simulink model "VC_GFM"  (R2023b)
settings: Solver=FixedStepAuto  StartTime=0.0  StopTime=1.5  RelTol=1e-3
InitFcn:
  | % 1. Récupérer les valeurs directement depuis le masque du Load Flow Bus4
  | V_amplitude_pu = str2double(get_param([bdroot '/Load Flow Bus4'], 'VLF'));
  | V_phase_deg    = str2double(get_param([bdroot '/Load Flow Bus4'], 'angleLF'));
  | 
  | % Assurez-vous que Vn est bien défini dans le modèle ou définissez-le ici
  | % Vn = 400; % (Exemple, à décommenter et adapter si Vn n'est pas connu du modèle)
  | 
  | % 2. Calculer et formater la chaîne de caractères pour le Sequence Analyzer
  | InInit_str = ['[', ...
  |     num2str(V_amplitude_pu * Vn * sqrt(2), '%.6f'), ', ', ...
  |     num2str(V_phase_deg, '%.6f'), ']'];
  | InInit_str2 = ['[', ...
  |     num2str((sqrt(2) * 0.5 * Sn_vcGFM) / (3 * V_amplitude_pu * Vn), '%.6f'), ', ', ...
  |     '0]'];
  | 
  | % 3. Injecter la valeur dans le Sequence Analyzer
  | set_param([bdroot '/Sequence Analyzer'], 'InInit', InInit_str);
  | set_param([bdroot '/Sequence Analyzer1'], 'InInit', InInit_str2);
undefined symbols (not defined in the file): delta_E, delta_Pvc, delta_theta_deg, enable_breaker, Lg, Rg, Tf, Ts
libraries: spsSequenceAnalyzerLib x2, spsThreePhaseParallelRLCLoadLib x2, GFM_Lib x1, Source_Lib x1, spsLoadFlowBusLib x1, spsPower3phInstantaneousLib x1, spsThreePhaseSeriesRLCBranchLib x1, spsThreePhaseVIMeasurementLib x1, spsThreePhaseBreakerLib x1, VSC_Lib x1, spspowerguiLib x1
settings Model: Creator=cyril  LastModifiedBy=pcstudentgele11

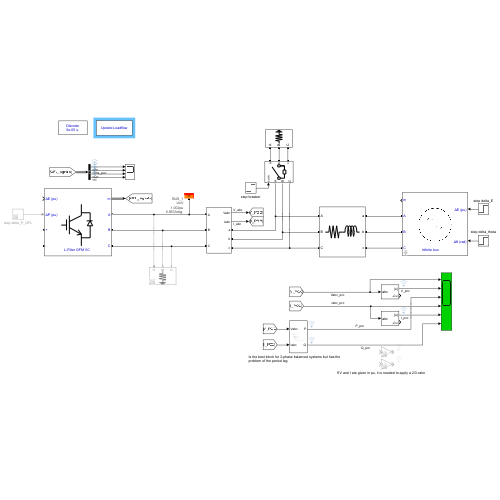
[thumbnail: Simulink's stored preview of the top-level diagram]
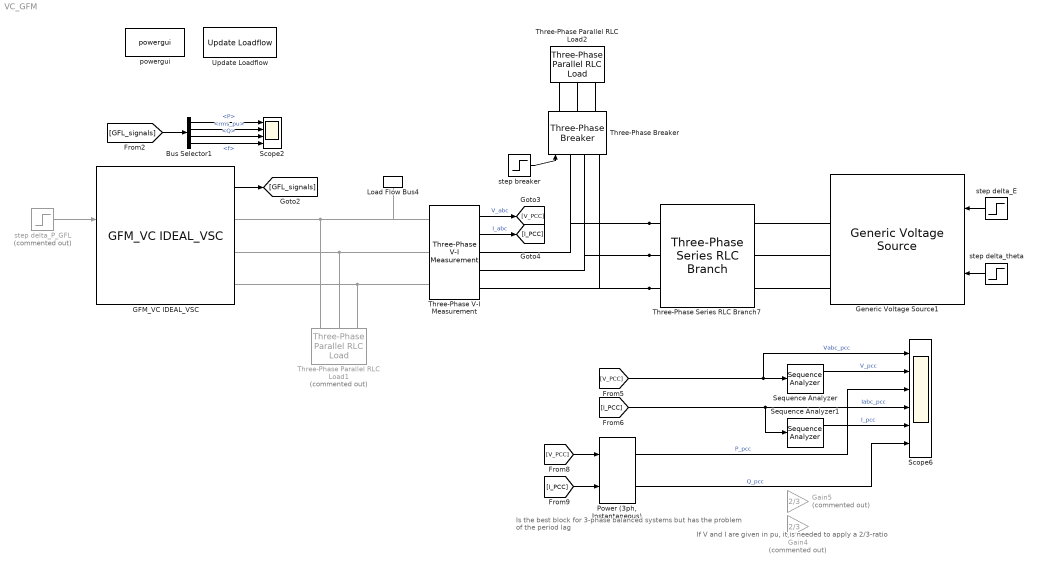
== system VC_GFM ==
  note: Is the best block for 3-phase balanced systems but has the problem of the period lag
  note: If V and I are given in pu, it is needed to apply a 2/3-ratio
  Bus Selector1 : BusSelector  OutputSignals=P,Vg.rms_pu,Q,f
  GFM_VC IDEAL_VSC : GFM_Lib/GFM_VC IDEAL_VSC  fn=fn  Sn=Sn_vcGFM  Pn=Sn_vcGFM  Udcn=Vdc  Output_Delay=Delayvc  Un1=Vnvsc  Un2=Un  Rt_pu=0.005  Lt_pu=0.15  Lm_pu=500  Rm_pu=500  DC_Link=Perfect DC Source  H_DC=inf  H_DC_sav=40  wn_PLL=50  zeta_PLL=1  Val_Freq_Support=on  R_percent=8  dLc_pu=0  Rv=Rvvc  W_TVR=W_TVRvc  I_max_pu=1.2  wn_I_max=300  I_Max_TVI_pu=1.2  DX_DR=5  Advanced=on  gainpopup=With Inertia  wn_Inertia_Less=10  Param_Inertia=PI  H_GFo=Hvc  zeta_GFo=ksivc  LFpopup=PQ  P0=0.5  Q0=0.00073  V0=1.0015  Theta0=0.95333
      settings: SourceProductName=VSC4SPS
  Gain4 : Gain  Commented=on  Gain=2/3
  Gain5 : Gain  Commented=on  Gain=2/3
  Generic Voltage Source1 : Source_Lib/Generic Voltage Source  SourceNature_str=INFINITE  fn=fn  Sn=Sng  Un=Un  H_s=5  DroopOnOff=on  R_percent=4  TN=1  TD=2  Time_Step=Ts  LFpopup=Swing  P0=-0.049915  Q0=0.00075769  V0=1  Theta0=0
      settings: SourceProductName=VSC4SPS
  Load Flow Bus4 : spsLoadFlowBusLib/Load Flow Bus  LConnTagsString=a  Phases=single  Connectors=on one side  ID=BUS_1  Vbase=Un  Vref=1  Vangle=0  VLF=1.002  VLFb=1  VLFc=1  angleLF=0.9533  angleLFb=0  angleLFc=0
  "Power (3ph, Instantaneous)" : spsPower3phInstantaneousLib/Power (3ph, Instantaneous)
  Scope2 : Scope  NumInputPorts=4
  Scope6 : Scope  NumInputPorts=6
  Sequence Analyzer : spsSequenceAnalyzerLib/Sequence Analyzer  Freq=50  n=1  seq=Positive  InInit=[327.251830, 0.953300]  Ts=0
  Sequence Analyzer1 : spsSequenceAnalyzerLib/Sequence Analyzer  Freq=50  n=1  seq=Positive  InInit=[10.185836, 0]  Ts=0
  Three-Phase Parallel RLC Load1 : spsThreePhaseParallelRLCLoadLib/Three-Phase Parallel RLC Load  Commented=on  LConnTagsString=A|B|C  Configuration=Y (grounded)  NominalVoltage=Un  Vabc=[1e3 1e3 1e3]  Vabcp=[1e3 1e3 1e3]  NominalFrequency=fn  UnbalancedPower=off  ActivePower=5  InductivePower=0  CapacitivePower=0  Pabc=[10e3 9e3 11e3]  QLabc=[100 90 110]  QCabc=[100 90 110]  Pabcp=[10e3 9e3 11e3]  QLabcp=[100 90 110]  QCabcp=[100 90 110]  Measurements=None  LoadType=constant Z
  Three-Phase Parallel RLC Load2 : spsThreePhaseParallelRLCLoadLib/Three-Phase Parallel RLC Load  LConnTagsString=A|B|C  Configuration=Y (grounded)  NominalVoltage=Un  Vabc=[1e3 1e3 1e3]  Vabcp=[1e3 1e3 1e3]  NominalFrequency=fn  UnbalancedPower=off  ActivePower=P_fault  InductivePower=Q_fault  CapacitivePower=0  Pabc=[10e3 9e3 11e3]  QLabc=[100 90 110]  QCabc=[100 90 110]  Pabcp=[10e3 9e3 11e3]  QLabcp=[100 90 110]  QCabcp=[100 90 110]  Measurements=None  LoadType=constant Z
  Three-Phase Series RLC Branch7 : spsThreePhaseSeriesRLCBranchLib/Three-Phase Series RLC Branch  LConnTagsString=A|B|C  RConnTagsString=A|B|C  BranchType=RL  Resistance=Rg  Inductance=Lg  Capacitance=1e-6  Measurements=None
  Three-Phase V-I Measurement : spsThreePhaseVIMeasurementLib/Three-Phase V-I Measurement  VoltageMeasurement=phase-to-ground  SetLabelV=off  LabelV=Vabc  Vpu=off  VpuLL=off  CurrentMeasurement=yes  SetLabelI=off  LabelI=Iabc  Ipu=off  Pbase=Sn  Vbase=U1n  OutputType=Complex  PhasorSimulation=off  PSBequivalent=0
  Three-Phase Breaker : spsThreePhaseBreakerLib/Three-Phase Breaker  InitialState=open  SwitchA=on  SwitchB=on  SwitchC=on  SwitchTimes=t_breaker  External=on  BreakerResistance=0.01  SnubberResistance=1e6  SnubberCapacitance=inf  Measurements=None
  Update Loadflow : VSC_Lib/Update Loadflow  ShowInLibBrowser=on
      settings: SourceProductName=VSC4SPS
  powergui : spspowerguiLib/powergui  Priority=1  SimulationMode=Discrete  SampleTime=Ts  frequency=60  Iterations=50  frequencyindice=50  Pbase=100000  ErrMax=1e-6  UnitsV=kV  UnitsW=MW  buscounter=14  FunctionMessages=off  echomessages=off  EnableUseOfTLC=off  CurrentSourceSwitches=off  DisableSnubberDevices=off  DisableRonSwitches=off  DisableVfSwitches=off  DisplayEquations=off  AutomaticDiscreteSolvers=off  SolverType=Tustin/Backward Euler (TBE)  Interpol=off  ExternalGateDelay=off  methode=off  Ts=100  x0status=blocks  SPID=on  SwTol=0  HookPort=off  NonlinearTolerance=1e-4  nMaxIteration=100  ContinueOnMaxIteration=off  RestoreLinks=warning  ResistiveCurrentMeasurement=off  Frange=[0:2:500]  Ylog=off  Xlog=on  ShowGrid=off  save=off  variable=ZData  structure=0  ZoomFFT=off  StartTime=0.0  cycles=1  DisplayStyle=1  fundamental=60  FreqAxis=off  MaxFrequency=1000  frequencyindicesteady=1  RmsSteady=1  display=off
  step breaker : Step  Time=Tf  After=enable_breaker  SampleTime=0
  step delta_E : Step  Time=Tf  After=delta_E  SampleTime=0
  step delta_P_GFL : Step  Commented=on  Time=0.0  After=delta_Pvc  SampleTime=0
  step delta_theta : Step  Time=Tf  After=delta_theta_deg*pi/180  SampleTime=0
  wires:
  Sequence Analyzer1/1 -> Scope6/5  "I_pcc"
  GFM_VC IDEAL_VSC/1 -> [GFL_signals]
  "Power (3ph, Instantaneous)"/2 -> Scope6/6  "Q_pcc"
  "Power (3ph, Instantaneous)"/1 -> Scope6/3  "P_pcc"
  step delta_theta/1 -> Generic Voltage Source1/2
  [V_PCC] -> Scope6/1, Sequence Analyzer/1  "Vabc_pcc"
  Bus Selector1/4 -> Scope2/4  "<f>"
  [I_PCC] -> "Power (3ph, Instantaneous)"/2
  [I_PCC] -> Scope6/4, Sequence Analyzer1/1  "Iabc_pcc"
  Sequence Analyzer/1 -> Scope6/2  "V_pcc"
  [GFL_signals] -> Bus Selector1/1
  Three-Phase V-I Measurement/1 -> [V_PCC]  "V_abc"
  step breaker/1 -> Three-Phase Breaker/1
  Three-Phase V-I Measurement/2 -> [I_PCC]  "I_abc"
  step delta_P_GFL/1 -> GFM_VC IDEAL_VSC/2
  Bus Selector1/1 -> Scope2/1  "<P>"
  Bus Selector1/2 -> Scope2/2  "<rms_pu>"
  Bus Selector1/3 -> Scope2/3  "<Q>"
  [V_PCC] -> "Power (3ph, Instantaneous)"/1
  step delta_E/1 -> Generic Voltage Source1/1
  connections:
  Three-Phase Parallel RLC Load1/LConn3 -- GFM_VC IDEAL_VSC/RConn3 -- Three-Phase V-I Measurement/LConn3
  Three-Phase Parallel RLC Load1/LConn1 -- Load Flow Bus4/LConn1 -- Three-Phase V-I Measurement/LConn1 -- GFM_VC IDEAL_VSC/RConn1
  Three-Phase Parallel RLC Load1/LConn2 -- GFM_VC IDEAL_VSC/RConn2 -- Three-Phase V-I Measurement/LConn2
  Three-Phase Series RLC Branch7/LConn2 -- Three-Phase V-I Measurement/RConn2 -- Three-Phase Breaker/LConn2
  Three-Phase Series RLC Branch7/LConn3 -- Three-Phase V-I Measurement/RConn3 -- Three-Phase Breaker/LConn3
  Three-Phase Series RLC Branch7/LConn1 -- Three-Phase V-I Measurement/RConn1 -- Three-Phase Breaker/LConn1
  Three-Phase Parallel RLC Load2/LConn1 -- Three-Phase Breaker/RConn1
  Three-Phase Breaker/RConn2 -- Three-Phase Parallel RLC Load2/LConn2
  Three-Phase Breaker/RConn3 -- Three-Phase Parallel RLC Load2/LConn3
  Three-Phase Series RLC Branch7/RConn1 -- Generic Voltage Source1/RConn1
  Three-Phase Series RLC Branch7/RConn3 -- Generic Voltage Source1/RConn3
  Three-Phase Series RLC Branch7/RConn2 -- Generic Voltage Source1/RConn2
